simulink model "VehicleDiagram"  (R2024b)
settings: Solver=ode4  StartTime=0  StopTime=T_end  FixedStep=Ts_plant  RelTol=1e-3
values from neighbouring files (symbols this model uses):
  brake_split = 0.6    [Model_Setup.m]
  C_rr = 0.015    [Model_Setup.m]
  CdA = 0.66    [Model_Setup.m]
  Cf = 2*19000    (= 38000)    [Model_Setup.m]
  Cr = 2*19000    (= 38000)    [Model_Setup.m]
  fin = struct('n_laps', 3, 'v_stop', 0.05, 't_hold', 0.5)    [Model_Setup.m]
  g = 9.81    [Model_Setup.m]    (also in mpc_qp.m = A*g;  g(:,k) = B)
  h = min(0.8, 0.35*n)    [Gorsellestirme.m]    (also in Model_Setup.m = 0.55; mpc_qp.m = [G'*Qb*F - p.Rd*u_prev*D'*e1; 0])
  Iz = 2250    [Model_Setup.m]
  L = 2.7    [Model_Setup.m]    (also in reference_path.m = sa(end))
  lf = evalin('base', 'lf')    [Gorsellestirme.m]    (also in Model_Setup.m = 1.35)
  lr = evalin('base', 'lr')    [Gorsellestirme.m]    (also in Model_Setup.m = 1.35)
  m = evalin('base', 'm')    [Gorsellestirme.m]    (also in Model_Setup.m = 1500; reference_path.m = max(ceil(Rc*abs(dlt(c))/h), 1))
  mpc_lat = struct('Np', 30, 'Q', diag([70 10 150 30]), 'R', 0, 'Rd', 1,      'ulim', deg2rad([-30 30]), 'dumax', 1.5*Ts_ctrl, 'isoft', 0, 'ws', 1,      'vx_floor', vx_floor, 'Cf', Cf, 'Cr', Cr, 'lf', lf, 'lr', lr, 'm', m, 'Iz', Iz)    [Model_Setup.m]
  mpc_lon = struct('Np', 30, 'Q', diag([150 10]), 'R', 0, 'Rd', 1,      'ulim', [-3 2], 'dumax', 2.5*Ts_ctrl, 'isoft', 2, 'ws', 1e4,      'ay_lim', 0.75*mu*g, 'lr', lr, 'lf', lf, 'Cf', Cf, 'Cr', Cr, 'm', m, 'rho_air', rho_air, 'CdA', CdA, 'C_rr', C_rr, 'g', g)    [Model_Setup.m]
  mu = 0.75    [Model_Setup.m]
  psi0 = ref.theta0    [Model_Setup.m]
  r0_init = 0    [Model_Setup.m]
  ref = evalin('base', 'ref')    [Gorsellestirme.m]    (also in Model_Setup.m = reference_path(waypoints, startPt, prm_ref); reference_path.m = struct('x', x, 'y', y, 'theta', theta, 'kappa', kappa,      )
  rho_air = 1.225    [Model_Setup.m]
  stop_enable = 1    [Model_Setup.m]
  theta_road = 0    [Model_Setup.m]
  Ts_ctrl = 0.02    [Model_Setup.m]
  vx0_init = ref.v(ref.idx0)    [Model_Setup.m]
  vx_floor = 1    [Model_Setup.m]
  vy0_init = 0    [Model_Setup.m]
  win_back = 20    [Model_Setup.m]
  win_fwd = 120    [Model_Setup.m]
  X0 = ref.x(ref.idx0)    [Model_Setup.m]
  Y0 = ref.y(ref.idx0)    [Model_Setup.m]
settings Model: Creator=kasimesen  LastModifiedBy=kasimesen
settings DataIOCC: SaveOutput=off  SaveTime=off
settings DebuggingCC: AlgebraicLoopMsg=error  ArtificialAlgebraicLoopMsg=error
settings ConfigComp: CovBoundaryAbsTol=1.0e-5

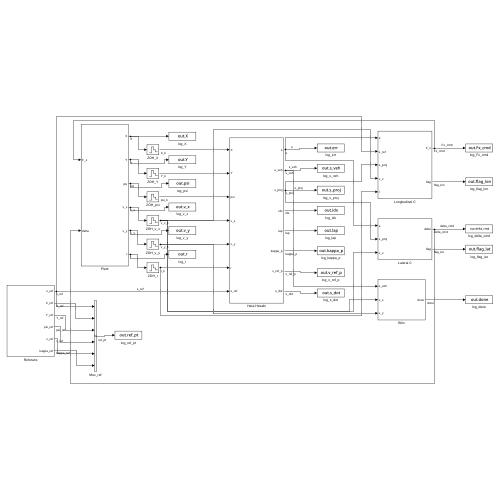
[thumbnail: Simulink's stored preview of the top-level diagram]
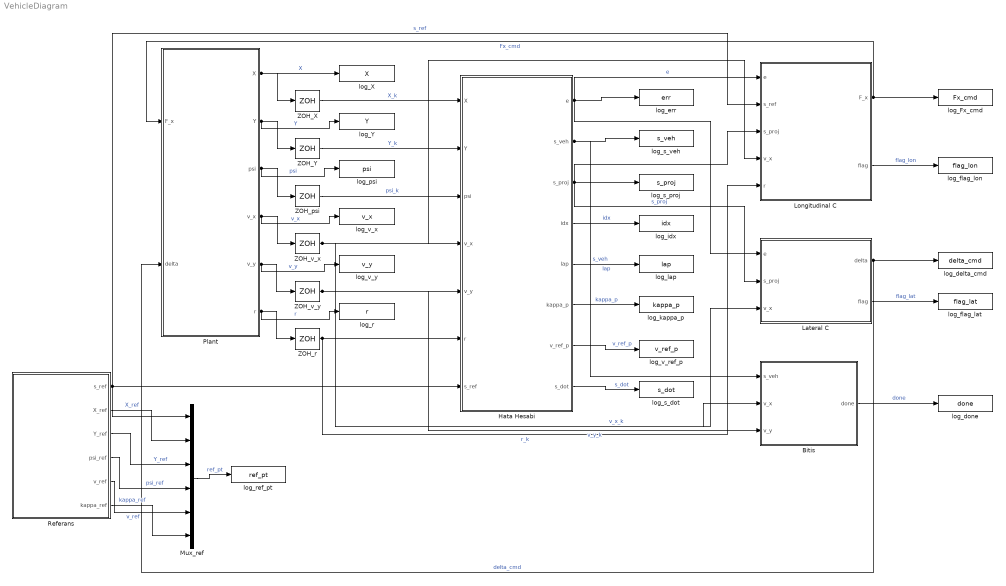
== system VehicleDiagram ==
  Bitis : Subsystem
  Hata Hesabi : Subsystem
  Lateral C : Subsystem
  Longitudinal C : Subsystem
  Mux_ref : Mux  Inputs=6
  Plant : Subsystem
  Referans : Subsystem
  ZOH_X : ZeroOrderHold  SampleTime=Ts_ctrl
  ZOH_Y : ZeroOrderHold  SampleTime=Ts_ctrl
  ZOH_psi : ZeroOrderHold  SampleTime=Ts_ctrl
  ZOH_r : ZeroOrderHold  SampleTime=Ts_ctrl
  ZOH_v_x : ZeroOrderHold  SampleTime=Ts_ctrl
  ZOH_v_y : ZeroOrderHold  SampleTime=Ts_ctrl
  log_Fx_cmd : ToWorkspace  VariableName=Fx_cmd  SaveFormat=Timeseries  SampleTime=-1
  log_X : ToWorkspace  VariableName=X  SaveFormat=Timeseries  SampleTime=-1
  log_Y : ToWorkspace  VariableName=Y  SaveFormat=Timeseries  SampleTime=-1
  log_delta_cmd : ToWorkspace  VariableName=delta_cmd  SaveFormat=Timeseries  SampleTime=-1
  log_done : ToWorkspace  VariableName=done  SaveFormat=Timeseries  SampleTime=-1
  log_err : ToWorkspace  VariableName=err  SaveFormat=Timeseries  SampleTime=-1
  log_flag_lat : ToWorkspace  VariableName=flag_lat  SaveFormat=Timeseries  SampleTime=-1
  log_flag_lon : ToWorkspace  VariableName=flag_lon  SaveFormat=Timeseries  SampleTime=-1
  log_idx : ToWorkspace  VariableName=idx  SaveFormat=Timeseries  SampleTime=-1
  log_kappa_p : ToWorkspace  VariableName=kappa_p  SaveFormat=Timeseries  SampleTime=-1
  log_lap : ToWorkspace  VariableName=lap  SaveFormat=Timeseries  SampleTime=-1
  log_psi : ToWorkspace  VariableName=psi  SaveFormat=Timeseries  SampleTime=-1
  log_r : ToWorkspace  VariableName=r  SaveFormat=Timeseries  SampleTime=-1
  log_ref_pt : ToWorkspace  VariableName=ref_pt  SaveFormat=Timeseries  SampleTime=-1
  log_s_dot : ToWorkspace  VariableName=s_dot  SaveFormat=Timeseries  SampleTime=-1
  log_s_proj : ToWorkspace  VariableName=s_proj  SaveFormat=Timeseries  SampleTime=-1
  log_s_veh : ToWorkspace  VariableName=s_veh  SaveFormat=Timeseries  SampleTime=-1
  log_v_ref_p : ToWorkspace  VariableName=v_ref_p  SaveFormat=Timeseries  SampleTime=-1
  log_v_x : ToWorkspace  VariableName=v_x  SaveFormat=Timeseries  SampleTime=-1
  log_v_y : ToWorkspace  VariableName=v_y  SaveFormat=Timeseries  SampleTime=-1
  wires:
  Plant/1(X) -> ZOH_X/1, log_X/1  "X"
  ZOH_X/1 -> Hata Hesabi/1(X)  "X_k"
  Plant/2(Y) -> ZOH_Y/1, log_Y/1  "Y"
  ZOH_Y/1 -> Hata Hesabi/2(Y)  "Y_k"
  Plant/3(psi) -> ZOH_psi/1, log_psi/1  "psi"
  ZOH_psi/1 -> Hata Hesabi/3(psi)  "psi_k"
  Plant/4(v_x) -> ZOH_v_x/1, log_v_x/1  "v_x"
  ZOH_v_x/1 -> Hata Hesabi/4(v_x), Longitudinal C/4(v_x), Lateral C/3(v_x), Bitis/2(v_x)  "v_x_k"
  Plant/5(v_y) -> ZOH_v_y/1, log_v_y/1  "v_y"
  ZOH_v_y/1 -> Hata Hesabi/5(v_y), Bitis/3(v_y)  "v_y_k"
  Plant/6(r) -> ZOH_r/1, log_r/1  "r"
  ZOH_r/1 -> Hata Hesabi/6(r), Longitudinal C/5(r)  "r_k"
  Referans/1(s_ref) -> Hata Hesabi/7(s_ref), Mux_ref/1, Longitudinal C/2(s_ref)  "s_ref"
  Referans/2(X_ref) -> Mux_ref/2  "X_ref"
  Referans/3(Y_ref) -> Mux_ref/3  "Y_ref"
  Referans/4(psi_ref) -> Mux_ref/4  "psi_ref"
  Referans/5(v_ref) -> Mux_ref/5  "v_ref"
  Referans/6(kappa_ref) -> Mux_ref/6  "kappa_ref"
  Mux_ref/1 -> log_ref_pt/1  "ref_pt"
  Hata Hesabi/1(e) -> log_err/1, Longitudinal C/1(e), Lateral C/1(e)  "e"
  Hata Hesabi/2(s_veh) -> log_s_veh/1, Bitis/1(s_veh)  "s_veh"
  Hata Hesabi/3(s_proj) -> log_s_proj/1, Longitudinal C/3(s_proj), Lateral C/2(s_proj)  "s_proj"
  Hata Hesabi/4(idx) -> log_idx/1  "idx"
  Hata Hesabi/5(lap) -> log_lap/1  "lap"
  Hata Hesabi/6(kappa_p) -> log_kappa_p/1  "kappa_p"
  Hata Hesabi/7(v_ref_p) -> log_v_ref_p/1  "v_ref_p"
  Hata Hesabi/8(s_dot) -> log_s_dot/1  "s_dot"
  Bitis/1(done) -> log_done/1  "done"
  Longitudinal C/1(F_x) -> log_Fx_cmd/1, Plant/1(F_x)  "Fx_cmd"
  Longitudinal C/2(flag) -> log_flag_lon/1  "flag_lon"
  Lateral C/1(delta) -> log_delta_cmd/1, Plant/2(delta)  "delta_cmd"
  Lateral C/2(flag) -> log_flag_lat/1  "flag_lat"

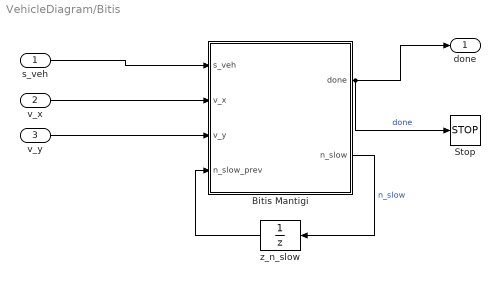
== system VehicleDiagram/Bitis ==
  s_veh : Inport
  v_x : Inport  Port=2
  v_y : Inport  Port=3
  Bitis Mantigi : MATLAB Function  TreatAsAtomicUnit=on
  Stop : Stop
  z_n_slow : UnitDelay  SampleTime=Ts_ctrl
  done : Outport
  wires:
  s_veh/1 -> Bitis Mantigi/1(s_veh)
  v_x/1 -> Bitis Mantigi/2(v_x)
  v_y/1 -> Bitis Mantigi/3(v_y)
  z_n_slow/1 -> Bitis Mantigi/4(n_slow_prev)
  Bitis Mantigi/2(n_slow) -> z_n_slow/1  "n_slow"
  Bitis Mantigi/1(done) -> done/1, Stop/1  "done"

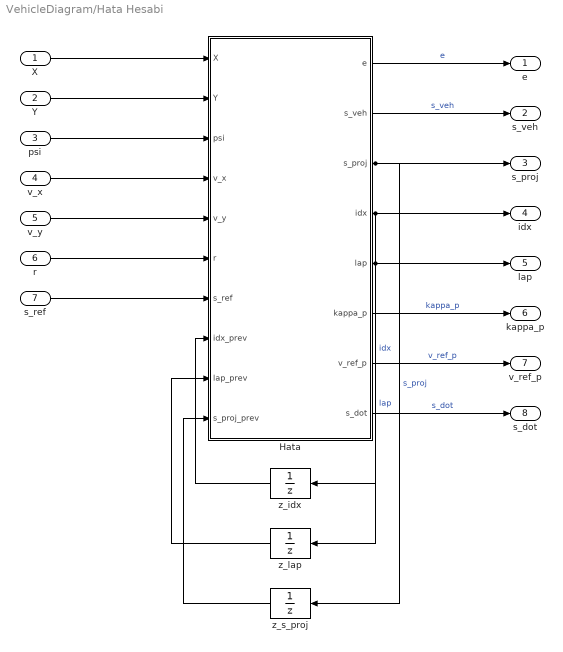
== system VehicleDiagram/Hata Hesabi ==
  X : Inport
  Y : Inport  Port=2
  psi : Inport  Port=3
  v_x : Inport  Port=4
  v_y : Inport  Port=5
  r : Inport  Port=6
  s_ref : Inport  Port=7
  Hata : MATLAB Function  TreatAsAtomicUnit=on
  z_idx : UnitDelay  SampleTime=Ts_ctrl
  z_lap : UnitDelay  SampleTime=Ts_ctrl
  z_s_proj : UnitDelay  SampleTime=Ts_ctrl
  e : Outport
  s_veh : Outport  Port=2
  s_proj : Outport  Port=3
  idx : Outport  Port=4
  lap : Outport  Port=5
  kappa_p : Outport  Port=6
  v_ref_p : Outport  Port=7
  s_dot : Outport  Port=8
  wires:
  X/1 -> Hata/1(X)
  Y/1 -> Hata/2(Y)
  psi/1 -> Hata/3(psi)
  v_x/1 -> Hata/4(v_x)
  v_y/1 -> Hata/5(v_y)
  r/1 -> Hata/6(r)
  s_ref/1 -> Hata/7(s_ref)
  Hata/1(e) -> e/1  "e"
  Hata/2(s_veh) -> s_veh/1  "s_veh"
  Hata/3(s_proj) -> s_proj/1, z_s_proj/1  "s_proj"
  Hata/4(idx) -> idx/1, z_idx/1  "idx"
  Hata/5(lap) -> lap/1, z_lap/1  "lap"
  Hata/6(kappa_p) -> kappa_p/1  "kappa_p"
  Hata/7(v_ref_p) -> v_ref_p/1  "v_ref_p"
  Hata/8(s_dot) -> s_dot/1  "s_dot"
  z_idx/1 -> Hata/8(idx_prev)
  z_lap/1 -> Hata/9(lap_prev)
  z_s_proj/1 -> Hata/10(s_proj_prev)

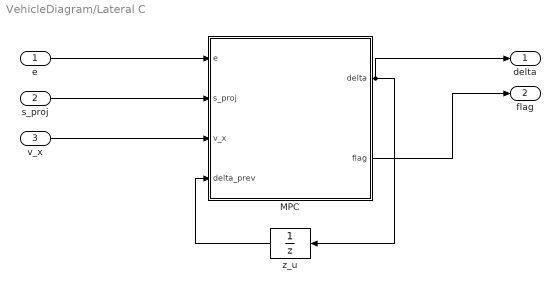
== system VehicleDiagram/Lateral C ==
  e : Inport
  s_proj : Inport  Port=2
  v_x : Inport  Port=3
  MPC : MATLAB Function  TreatAsAtomicUnit=on
  z_u : UnitDelay  SampleTime=Ts_ctrl
  delta : Outport
  flag : Outport  Port=2
  wires:
  e/1 -> MPC/1(e)
  s_proj/1 -> MPC/2(s_proj)
  v_x/1 -> MPC/3(v_x)
  z_u/1 -> MPC/4(delta_prev)
  MPC/1(delta) -> z_u/1, delta/1
  MPC/2(flag) -> flag/1

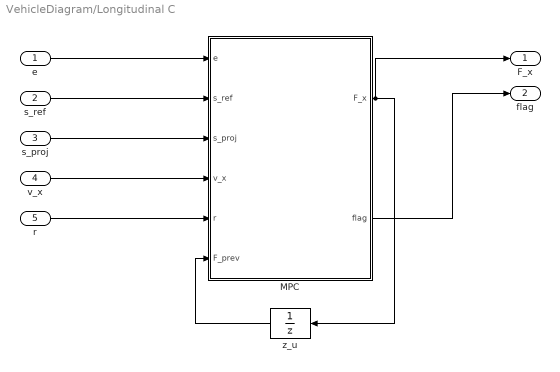
== system VehicleDiagram/Longitudinal C ==
  e : Inport
  s_ref : Inport  Port=2
  s_proj : Inport  Port=3
  v_x : Inport  Port=4
  r : Inport  Port=5
  MPC : MATLAB Function  TreatAsAtomicUnit=on
  z_u : UnitDelay  SampleTime=Ts_ctrl
  F_x : Outport
  flag : Outport  Port=2
  wires:
  e/1 -> MPC/1(e)
  s_ref/1 -> MPC/2(s_ref)
  s_proj/1 -> MPC/3(s_proj)
  v_x/1 -> MPC/4(v_x)
  r/1 -> MPC/5(r)
  z_u/1 -> MPC/6(F_prev)
  MPC/1(F_x) -> z_u/1, F_x/1
  MPC/2(flag) -> flag/1

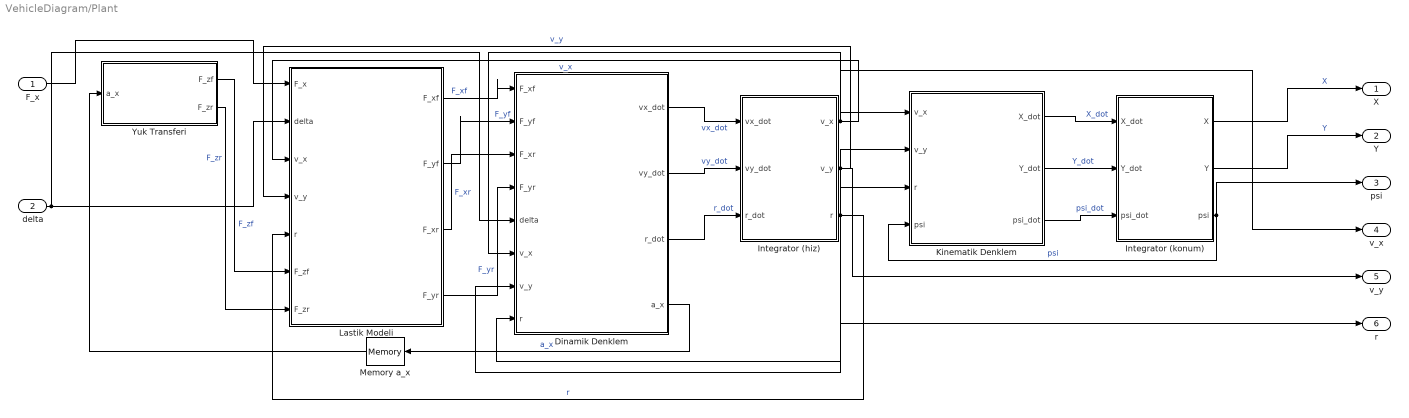
== system VehicleDiagram/Plant ==
  F_x : Inport
  delta : Inport  Port=2
  Dinamik Denklem : MATLAB Function  TreatAsAtomicUnit=on
  Integrator (hiz) : Subsystem
  Integrator (konum) : Subsystem
  Kinematik Denklem : MATLAB Function  TreatAsAtomicUnit=on
  Lastik Modeli : MATLAB Function  TreatAsAtomicUnit=on
  Memory a_x : Memory
  Yuk Transferi : MATLAB Function  TreatAsAtomicUnit=on
  X : Outport
  Y : Outport  Port=2
  psi : Outport  Port=3
  v_x : Outport  Port=4
  v_y : Outport  Port=5
  r : Outport  Port=6
  wires:
  Dinamik Denklem/4(a_x) -> Memory a_x/1  "a_x"
  Memory a_x/1 -> Yuk Transferi/1(a_x)
  F_x/1 -> Lastik Modeli/1(F_x)
  delta/1 -> Lastik Modeli/2(delta), Dinamik Denklem/5(delta)
  Yuk Transferi/1(F_zf) -> Lastik Modeli/6(F_zf)  "F_zf"
  Yuk Transferi/2(F_zr) -> Lastik Modeli/7(F_zr)  "F_zr"
  Lastik Modeli/1(F_xf) -> Dinamik Denklem/1(F_xf)  "F_xf"
  Lastik Modeli/2(F_yf) -> Dinamik Denklem/2(F_yf)  "F_yf"
  Lastik Modeli/3(F_xr) -> Dinamik Denklem/3(F_xr)  "F_xr"
  Lastik Modeli/4(F_yr) -> Dinamik Denklem/4(F_yr)  "F_yr"
  Dinamik Denklem/1(vx_dot) -> Integrator (hiz)/1(vx_dot)  "vx_dot"
  Integrator (hiz)/1(v_x) -> Lastik Modeli/3(v_x), Dinamik Denklem/6(v_x), Kinematik Denklem/1(v_x), v_x/1  "v_x"
  Kinematik Denklem/1(X_dot) -> Integrator (konum)/1(X_dot)  "X_dot"
  Dinamik Denklem/2(vy_dot) -> Integrator (hiz)/2(vy_dot)  "vy_dot"
  Integrator (hiz)/2(v_y) -> Lastik Modeli/4(v_y), Dinamik Denklem/7(v_y), Kinematik Denklem/2(v_y), v_y/1  "v_y"
  Kinematik Denklem/2(Y_dot) -> Integrator (konum)/2(Y_dot)  "Y_dot"
  Dinamik Denklem/3(r_dot) -> Integrator (hiz)/3(r_dot)  "r_dot"
  Integrator (hiz)/3(r) -> Lastik Modeli/5(r), Dinamik Denklem/8(r), Kinematik Denklem/3(r), r/1  "r"
  Kinematik Denklem/3(psi_dot) -> Integrator (konum)/3(psi_dot)  "psi_dot"
  Integrator (konum)/3(psi) -> Kinematik Denklem/4(psi), psi/1  "psi"
  Integrator (konum)/1(X) -> X/1  "X"
  Integrator (konum)/2(Y) -> Y/1  "Y"

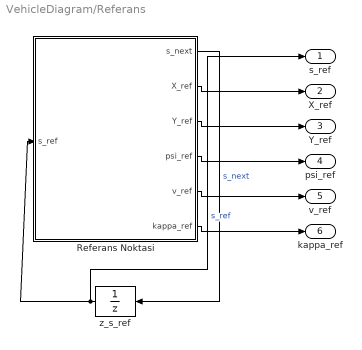
== system VehicleDiagram/Referans ==
  Referans Noktasi : MATLAB Function  TreatAsAtomicUnit=on
  z_s_ref : UnitDelay  InitialCondition=ref.s0  SampleTime=Ts_ctrl
  s_ref : Outport
  X_ref : Outport  Port=2
  Y_ref : Outport  Port=3
  psi_ref : Outport  Port=4
  v_ref : Outport  Port=5
  kappa_ref : Outport  Port=6
  wires:
  z_s_ref/1 -> Referans Noktasi/1(s_ref), s_ref/1  "s_ref"
  Referans Noktasi/1(s_next) -> z_s_ref/1  "s_next"
  Referans Noktasi/2(X_ref) -> X_ref/1
  Referans Noktasi/3(Y_ref) -> Y_ref/1
  Referans Noktasi/4(psi_ref) -> psi_ref/1
  Referans Noktasi/5(v_ref) -> v_ref/1
  Referans Noktasi/6(kappa_ref) -> kappa_ref/1

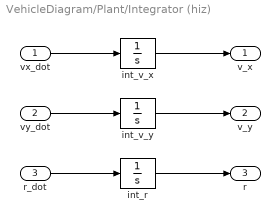
== system VehicleDiagram/Plant/Integrator (hiz) ==
  vx_dot : Inport
  vy_dot : Inport  Port=2
  r_dot : Inport  Port=3
  int_r : Integrator  InitialCondition=r0_init
  int_v_x : Integrator  InitialCondition=vx0_init  LimitOutput=on  LowerSaturationLimit=0
  int_v_y : Integrator  InitialCondition=vy0_init
  v_x : Outport
  v_y : Outport  Port=2
  r : Outport  Port=3
  wires:
  vx_dot/1 -> int_v_x/1
  int_v_x/1 -> v_x/1
  vy_dot/1 -> int_v_y/1
  int_v_y/1 -> v_y/1
  r_dot/1 -> int_r/1
  int_r/1 -> r/1

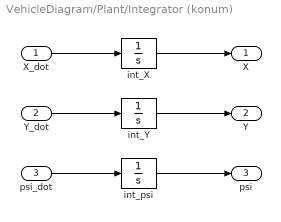
== system VehicleDiagram/Plant/Integrator (konum) ==
  X_dot : Inport
  Y_dot : Inport  Port=2
  psi_dot : Inport  Port=3
  int_X : Integrator  InitialCondition=X0
  int_Y : Integrator  InitialCondition=Y0
  int_psi : Integrator  InitialCondition=psi0
  X : Outport
  Y : Outport  Port=2
  psi : Outport  Port=3
  wires:
  X_dot/1 -> int_X/1
  int_X/1 -> X/1
  Y_dot/1 -> int_Y/1
  int_Y/1 -> Y/1
  psi_dot/1 -> int_psi/1
  int_psi/1 -> psi/1

== matlab function VehicleDiagram/Referans/Referans Noktasi ==
  data: s_ref input; s_next output size=1; X_ref output size=1; Y_ref output size=1; psi_ref output size=1; v_ref output size=1; kappa_ref output size=1; ref parameter; Ts_ctrl parameter
function [s_next, X_ref, Y_ref, psi_ref, v_ref, kappa_ref] = fcn(s_ref, ref, Ts_ctrl)
% Referans Noktasi: s_ref[k+1] = s_ref[k] + v_ref(s_ref[k] mod L) Ts_ctrl
% (s_ref acilmis, baslangic ref.s0 = z_s_ref IC); s_ref noktasinda yolun
% konumu, yonu, hizi ve egriligi (lineer ara deger, yon sarma farkiyla).
s_next    = s_ref + periodic_interp(ref.v, s_ref, ref.ds)*Ts_ctrl;
X_ref     = periodic_interp(ref.x, s_ref, ref.ds);
Y_ref     = periodic_interp(ref.y, s_ref, ref.ds);
v_ref     = periodic_interp(ref.v, s_ref, ref.ds);
kappa_ref = periodic_interp(ref.kappa, s_ref, ref.ds);
N = numel(ref.theta);
u = s_ref/ref.ds;  j = floor(u);  t = u - j;
a = mod(j, N) + 1;  b = mod(j + 1, N) + 1;
dth = mod(ref.theta(b) - ref.theta(a) + pi, 2*pi) - pi;
psi_ref = mod(ref.theta(a) + t*dth + pi, 2*pi) - pi;

== matlab function VehicleDiagram/Hata Hesabi/Hata ==
  data: X input; Y input; psi input; v_x input; v_y input; r input; e output size=6; s_ref input; idx_prev input; lap_prev input; s_proj_prev input; s_veh output size=1; s_proj output size=1; idx output size=1; lap output size=1; kappa_p output size=1; v_ref_p output size=1; s_dot output size=1; ref parameter; win_fwd parameter; win_back parameter
function [e, s_veh, s_proj, idx, lap, kappa_p, v_ref_p, s_dot] = fcn(X, Y, psi, v_x, v_y, r, s_ref, idx_prev, lap_prev, s_proj_prev, ref, win_fwd, win_back)
% Hata: arac durumu X, Y, psi, v_x, v_y, r (ZOH), s_ref acilmis. ref_error (Rajamani 2.5).
% e = [e_x; e_y; e_psi; e_x_dot; e_y_dot; e_psi_dot].
[e_x, e_y, e_psi, e_x_dot, e_y_dot, e_psi_dot, s_veh, s_proj, idx, lap, ~, v_ref_p, kappa_p, ~, s_dot] = ...
    ref_error(X, Y, psi, v_x, v_y, r, s_ref, idx_prev, lap_prev, s_proj_prev, ...
              ref, win_fwd, win_back);
e = [e_x; e_y; e_psi; e_x_dot; e_y_dot; e_psi_dot];
end

%% ======================================================================
function [e_x, e_y, e_psi, e_x_dot, e_y_dot, e_psi_dot, s_veh, s_proj, idx, lap, ...
          v_ref_s, v_ref_p, kappa_p, theta_p, s_dot] = ref_error( ...
          X, Y, psi, v_x, v_y, r, s_ref, idx_prev, lap_prev, s_proj_prev, ref, win_fwd, win_back)
%REF_ERROR  Yola izdusum ve takip hatalari (S2, Rajamani 2.5 isaret kurali).
%   Girisler: arac durumu X, Y, psi, v_x, v_y, r; acilmis s_ref; geri
%   besleme durumlari idx_prev (< 1 = ilk adim, tum yolda arama), lap_prev,
%   s_proj_prev; ref = reference_path ciktisi; pencere win_fwd / win_back
%   (dugum sayisi, varsayilan 120 / 20).
%   1) En yakin dugum: ilk adimda global, sonra idx_prev - win_back ...
%      idx_prev + win_fwd penceresi (mod N).
%   2) Komsu iki segmente dik izdusum, yakin olan secilir; sonra izdusum
%      noktasi, ara degerli teget theta_p'ye dik olacak sekilde 3 Newton
%      adimiyla duzeltilir (e_x, s icin; buyuk e_y'de kiris yonu hatasini
%      kaldirir). s_proj surekli, [0, L) (kayan noktada mod sonucu L'ye
%      esit olabilir; path_at bunu son segmentin t = 1 ucu olarak okur,
%      tur sayaci etkilenmez).
%   3) e_y = -(X-Xp) sin(theta_p) + (Y-Yp) cos(theta_p)   (sola pozitif)
%          + kappa_p t (1-t) ds^2 / 2   (kiris -> yerel yay duzeltmesi)
%      e_psi = wrap(psi - theta_p)
%      e_y_dot = v_x sin(e_psi) + v_y cos(e_psi)
%      s_dot = (v_x cos(e_psi) - v_y sin(e_psi)) / (1 - kappa_p e_y)
%      e_psi_dot = r - kappa_p s_dot
%   4) Tur: s_proj - s_proj_prev < -L/2 -> lap+1, > L/2 -> lap-1. Ilk adimda
%      lap = round((s_ref - s_proj)/L) (s_veh, s_ref'e en yakin tur).
%      s_veh = s_proj + lap L;  e_x = s_ref - s_veh (+ = arac geride);
%      e_x_dot = v_ref(s_ref) - s_dot.
%   Yoldan uzak arac icin de sonlu deger doner: Newton adiminda ve s_dot
%   paydasinda 1 - kappa_p e_y >= 0.05 tabani (taban yalniz egrilik
%   merkezine 0.05 R'den yakin, fiziksel olmayan bolgede devreye girer).
%#codegen
N  = numel(ref.x);
ds = ref.ds;
L  = ref.L;

%% 1) En yakin dugum
ip   = round(idx_prev);
best = inf;
idx  = 1;
if ip < 1
    for j = 1:N
        d2 = (ref.x(j) - X)^2 + (ref.y(j) - Y)^2;
        if d2 < best, best = d2; idx = j; end
    end
else
    for k = -win_back:win_fwd
        j  = mod(ip - 1 + k, N) + 1;
        d2 = (ref.x(j) - X)^2 + (ref.y(j) - Y)^2;
        if d2 < best, best = d2; idx = j; end
    end
end

%% 2) Komsu segmentlere izdusum + Newton duzeltmesi
ia = mod(idx - 2, N) + 1;
ib = mod(idx, N) + 1;
[t1, d1] = seg_proj(ref.x(ia), ref.y(ia), ref.x(idx), ref.y(idx), X, Y);
[t2, d2] = seg_proj(ref.x(idx), ref.y(idx), ref.x(ib), ref.y(ib), X, Y);
if d1 < d2
    s_p = (ia - 1 + t1) * ds;
else
    s_p = (idx - 1 + t2) * ds;
end
s_p = mod(s_p, L);
for it = 1:3
    [xp, yp, thp, kp] = path_at(ref, s_p);
    dx  = X - xp;
    dy  = Y - yp;
    eyt = -dx*sin(thp) + dy*cos(thp);
    stp = (dx*cos(thp) + dy*sin(thp)) / max(1 - kp*eyt, 0.05);
    stp = min(max(stp, -ds), ds);
    s_p = mod(s_p + stp, L);
end
s_proj = s_p;
[xp, yp, theta_p, kappa_p, tp] = path_at(ref, s_proj);

%% 3) Hatalar
% kiris yerine yerel yay: egri, kirisin kappa_p t(1-t) ds^2/2 sagindadir
e_y   = -(X - xp)*sin(theta_p) + (Y - yp)*cos(theta_p) + kappa_p*tp*(1 - tp)*ds^2/2;
e_psi = wrap_pi(psi - theta_p);
e_y_dot   = v_x*sin(e_psi) + v_y*cos(e_psi);
s_dot     = (v_x*cos(e_psi) - v_y*sin(e_psi)) / max(1 - kappa_p*e_y, 0.05);
e_psi_dot = r - kappa_p*s_dot;

%% 4) Tur sayaci ve boyuna hata
if ip < 1
    lap = round((s_ref - s_proj) / L);
else
    lap = lap_prev;
    if s_proj - s_proj_prev < -L/2
        lap = lap + 1;
    elseif s_proj - s_proj_prev > L/2
        lap = lap - 1;
    end
end
s_veh   = s_proj + lap*L;
e_x     = s_ref - s_veh;
v_ref_s = periodic_interp(ref.v, s_ref, ds);
v_ref_p = periodic_interp(ref.v, s_proj, ds);
e_x_dot = v_ref_s - s_dot;
end

%% ======================================================================
function [t, d2] = seg_proj(xa, ya, xb, yb, X, Y)
% a -> b segmentine dik izdusum parametresi t in [0, 1] ve uzaklik karesi
ux = xb - xa;  uy = yb - ya;
t  = ((X - xa)*ux + (Y - ya)*uy) / max(ux*ux + uy*uy, eps);
t  = min(max(t, 0), 1);
d2 = (X - xa - t*ux)^2 + (Y - ya - t*uy)^2;
end

function [xp, yp, thp, kp, t] = path_at(ref, s)
% s in [0, L) noktasinda konum, yon (wrap'li) ve egrilik, lineer ara deger;
% t = segment ici parametre
N  = numel(ref.x);
u  = s / ref.ds;
j  = min(floor(u), N - 1);
t  = u - j;
a  = j + 1;
b  = mod(j + 1, N) + 1;
xp  = ref.x(a) + t*(ref.x(b) - ref.x(a));
yp  = ref.y(a) + t*(ref.y(b) - ref.y(a));
thp = wrap_pi(ref.theta(a) + t*wrap_pi(ref.theta(b) - ref.theta(a)));
kp  = ref.kappa(a) + t*(ref.kappa(b) - ref.kappa(a));
end

function a = wrap_pi(a)
a = mod(a + pi, 2*pi) - pi;
end

== matlab function VehicleDiagram/Bitis/Bitis Mantigi ==
  data: s_veh input; done output size=1; v_x input; v_y input; n_slow_prev input; n_slow output size=1; stop_enable parameter; ref parameter; fin parameter; Ts_ctrl parameter
function [done, n_slow] = fcn(s_veh, v_x, v_y, n_slow_prev, stop_enable, ref, fin, Ts_ctrl)
% Bitis Mantigi: tur (s_veh - s0 >= n_laps L) ya da t_hold boyunca
% hypot(v_x, v_y) < v_stop; stop_enable = 0 iken hic bitmez (ref_done).
[done, n_slow] = ref_done(s_veh, v_x, v_y, n_slow_prev, stop_enable, ref, fin, Ts_ctrl);
end

%% ======================================================================
function [done, n_slow] = ref_done(s_veh, v_x, v_y, n_slow_prev, stop_enable, ref, fin, Ts)
%REF_DONE  Bitis mantigi (S2).
%   [done, n_slow] = ref_done(s_veh, v_x, v_y, n_slow_prev, stop_enable, ref, fin, Ts)
%   fin: n_laps, v_stop, t_hold. Ts: ornekleme suresi (Simulink'te Ts_ctrl;
%   Referans Noktasi ile ayni tek kaynak).
%   n_slow : hypot(v_x, v_y) < v_stop olan ardisik ornek sayisi (geri
%            besleme, baslangic 0).
%   done = stop_enable VE ( s_veh - s0 >= n_laps*L
%                           VEYA (n_slow - 1)*Ts >= t_hold ).
%   Ilk yavas ornek k0 ise durma olcutu k0 + t_hold/Ts adiminda tetiklenir
%   (arac en az t_hold boyunca kesintisiz yavas). stop_enable = 0 iken done
%   hic 1 olmaz; n_slow yine sayilir.
%#codegen
if hypot(v_x, v_y) < fin.v_stop
    n_slow = n_slow_prev + 1;
else
    n_slow = 0;
end
lap_ok  = s_veh - ref.s0 >= fin.n_laps * ref.L;
stop_ok = n_slow >= 1 && (n_slow - 1) * Ts >= fin.t_hold - 1e-9;
done = double(stop_enable ~= 0 && (lap_ok || stop_ok));
end

== matlab function VehicleDiagram/Lateral C/MPC ==
  data: e input; delta output size=1; s_proj input; v_x input; delta_prev input; flag output size=1; ref parameter; mpc_lat parameter; Ts_ctrl parameter
function [delta, flag] = fcn(e, s_proj, v_x, delta_prev, ref, mpc_lat, Ts_ctrl)
% Lateral C: yanal MPC (lat_mpc, MATLAB'da calisir; quadprog).
coder.extrinsic('lat_mpc');
delta = 0;  flag = 0;
[delta, flag] = lat_mpc(e, s_proj, v_x, delta_prev, ref, mpc_lat, Ts_ctrl);

== matlab function VehicleDiagram/Longitudinal C/MPC ==
  data: e input; F_x output size=1; s_ref input; s_proj input; v_x input; r input; F_prev input; flag output size=1; ref parameter; mpc_lon parameter; Ts_ctrl parameter
function [F_x, flag] = fcn(e, s_ref, s_proj, v_x, r, F_prev, ref, mpc_lon, Ts_ctrl)
% Longitudinal C: boyuna MPC (lon_mpc, MATLAB'da calisir; quadprog).
coder.extrinsic('lon_mpc');
F_x = 0;  flag = 0;
[F_x, flag] = lon_mpc(e(1), s_ref, s_proj, v_x, v_x*r, F_prev, ref, mpc_lon, Ts_ctrl);

== matlab function VehicleDiagram/Plant/Lastik Modeli ==
  data: F_x input; F_xf output; delta input; v_x input; v_y input; r input; F_zf input; F_zr input; F_yf output; F_xr output; F_yr output; lf parameter; lr parameter; Cf parameter; Cr parameter; mu parameter; vx_floor parameter; brake_split parameter
function [F_xf, F_yf, F_xr, F_yr] = fcn(F_x, delta, v_x, v_y, r, F_zf, F_zr, lf, lr, Cf, Cr, mu, vx_floor, brake_split)
% Lastik Modeli: kuvvetler teker cercevesinde, aks basina (iki teker toplu).
% Itis yalniz arkadan; fren brake_split ile on/arka.
if F_x >= 0
    F_xf = 0;
    F_xr = F_x;
else
    F_xf = brake_split*F_x;
    F_xr = (1 - brake_split)*F_x;
end
% surtunme cemberi: once boyuna kirpilir, kalan pay yanal tavandir
F_xf = min(max(F_xf, -mu*F_zf), mu*F_zf);
F_xr = min(max(F_xr, -mu*F_zr), mu*F_zr);
% kayma acilari (S1 notlar), bolme tabani vx_floor
vx_hat = max(v_x, vx_floor);
a_f = delta - atan((v_y + lf*r)/vx_hat);
a_r = -atan((v_y - lr*r)/vx_hat);
F_yf = dugoff(a_f, Cf, sqrt(max((mu*F_zf)^2 - F_xf^2, 0)));
F_yr = dugoff(a_r, Cr, sqrt(max((mu*F_zr)^2 - F_xr^2, 0)));
end

function F = dugoff(a, C, Fmax)
% Yanal Dugoff (Rajamani 13, kappa yok), S = C|tan a|: 2S <= Fmax dogrusal,
% degilse doymus. Fmax = 0 iken F = 0 (S = 0 dogrusal kol, S > 0 doymus kol).
S = C*abs(tan(a));
if 2*S <= Fmax
    F = C*tan(a);
else
    F = sign(a)*Fmax*(1 - Fmax/(4*S));
end
end

== matlab function VehicleDiagram/Plant/Yuk Transferi ==
  data: a_x input; F_zf output; F_zr output; m parameter; g parameter; lf parameter; lr parameter; L parameter; h parameter
function [F_zf, F_zr] = fcn(a_x, m, g, lf, lr, L, h)
% Yuk Transferi: aks dusey yukleri (>= 0); a_x govde boyuna ivmesi,
% Memory a_x uzerinden bir adim (Ts_plant) gecikmeli.
F_zf = max((m*g*lr - m*a_x*h)/L, 0);
F_zr = max((m*g*lf + m*a_x*h)/L, 0);

== matlab function VehicleDiagram/Plant/Dinamik Denklem ==
  data: F_xf input; vx_dot output; F_yf input; F_xr input; F_yr input; delta input; v_x input; v_y input; r input; vy_dot output; r_dot output; a_x output; m parameter; Iz parameter; lf parameter; lr parameter; rho_air parameter; CdA parameter; C_rr parameter; g parameter; theta_road parameter
function [vx_dot, vy_dot, r_dot, a_x] = fcn(F_xf, F_yf, F_xr, F_yr, delta, v_x, v_y, r, m, Iz, lf, lr, rho_air, CdA, C_rr, g, theta_road)
% Dinamik Denklem: tam form govde denklemleri (Rajamani 2.3), lastik
% kuvvetleri (teker cercevesi, aks basina) Lastik Modeli'nden gelir.
% Direnc: hava + yuvarlanma + egim (S1; v_x >= 0).
F_res = 0.5*rho_air*CdA*v_x^2 + C_rr*m*g*cos(theta_road) + m*g*sin(theta_road);
vx_dot = (F_xf*cos(delta) - F_yf*sin(delta) + F_xr - F_res)/m + v_y*r;
vy_dot = (F_yf*cos(delta) + F_xf*sin(delta) + F_yr)/m - v_x*r;
r_dot  = (lf*(F_yf*cos(delta) + F_xf*sin(delta)) - lr*F_yr)/Iz;
a_x    = vx_dot - v_y*r;   % govde boyuna ivmesi (yuk transferi icin)

== matlab function VehicleDiagram/Plant/Kinematik Denklem ==
  data: v_x input; X_dot output; v_y input; r input; psi input; Y_dot output; psi_dot output
function [X_dot, Y_dot, psi_dot] = fcn(v_x, v_y, r, psi)
% Kinematik Denklem: govde hizlarindan global konum turevleri.
X_dot   = v_x*cos(psi) - v_y*sin(psi);
Y_dot   = v_x*sin(psi) + v_y*cos(psi);
psi_dot = r;
